simulink model "s_b16a4x32kf"  (R2018a)
settings: Solver=VariableStepDiscrete  StartTime=0.0  StopTime=1000  RelTol=1e-3
undefined symbols (not defined in the file): fft_stages, n_bits_ants, n_bits_xengs
libraries: xbsIndex_r4 x23740, casper_library_misc x48, casper_library_delays x8, xps_library x4, casper_library_scopes x1
(part 93 of 219)

== system s_b16a4x32kf/sys2/pkt_reord/munge/split ==
  bus_in : Inport
  reinterpret{1..9} (9 alike) : xbsIndex_r4/Reinterpret  force_arith_type=on  arith_type=Unsigned  force_bin_pt=on  bin_pt=0  block_type=reinterpret
  slice1 : xbsIndex_r4/Slice  nbits=32  boolean_output=off  mode=Upper Bit Location + Width  bit1=-225  base1=MSB of Input  bit0=0  base0=LSB of Input  dbl_ovrd=off  block_type=slice
  slice2 : xbsIndex_r4/Slice  nbits=32  boolean_output=off  mode=Upper Bit Location + Width  bit1=-193  base1=MSB of Input  bit0=0  base0=LSB of Input  dbl_ovrd=off  block_type=slice
  slice3 : xbsIndex_r4/Slice  nbits=32  boolean_output=off  mode=Upper Bit Location + Width  bit1=-161  base1=MSB of Input  bit0=0  base0=LSB of Input  dbl_ovrd=off  block_type=slice
  slice4 : xbsIndex_r4/Slice  nbits=32  boolean_output=off  mode=Upper Bit Location + Width  bit1=-129  base1=MSB of Input  bit0=0  base0=LSB of Input  dbl_ovrd=off  block_type=slice
  slice5 : xbsIndex_r4/Slice  nbits=32  boolean_output=off  mode=Upper Bit Location + Width  bit1=-97  base1=MSB of Input  bit0=0  base0=LSB of Input  dbl_ovrd=off  block_type=slice
  slice6 : xbsIndex_r4/Slice  nbits=32  boolean_output=off  mode=Upper Bit Location + Width  bit1=-65  base1=MSB of Input  bit0=0  base0=LSB of Input  dbl_ovrd=off  block_type=slice
  slice7 : xbsIndex_r4/Slice  nbits=32  boolean_output=off  mode=Upper Bit Location + Width  bit1=-33  base1=MSB of Input  bit0=0  base0=LSB of Input  dbl_ovrd=off  block_type=slice
  slice8 : xbsIndex_r4/Slice  nbits=32  boolean_output=off  mode=Upper Bit Location + Width  bit1=-1  base1=MSB of Input  bit0=0  base0=LSB of Input  dbl_ovrd=off  block_type=slice
  slice9 : xbsIndex_r4/Slice  nbits=1  boolean_output=off  mode=Upper Bit Location + Width  bit1=0  base1=MSB of Input  bit0=0  base0=LSB of Input  dbl_ovrd=off  block_type=slice
  msb_out9 : Outport
  out8 : Outport  Port=2
  out7 : Outport  Port=3
  out6 : Outport  Port=4
  out5 : Outport  Port=5
  out4 : Outport  Port=6
  out3 : Outport  Port=7
  out2 : Outport  Port=8
  lsb_out1 : Outport  Port=9
  wires:
  bus_in/1 -> slice9/1, slice8/1, slice7/1, slice6/1, slice5/1, slice4/1, slice3/1, slice2/1, slice1/1
  slice9/1 -> reinterpret9/1
  reinterpret9/1 -> msb_out9/1
  slice8/1 -> reinterpret8/1
  reinterpret8/1 -> out8/1
  slice7/1 -> reinterpret7/1
  reinterpret7/1 -> out7/1
  slice6/1 -> reinterpret6/1
  reinterpret6/1 -> out6/1
  slice5/1 -> reinterpret5/1
  reinterpret5/1 -> out5/1
  slice4/1 -> reinterpret4/1
  reinterpret4/1 -> out4/1
  slice3/1 -> reinterpret3/1
  reinterpret3/1 -> out3/1
  slice2/1 -> reinterpret2/1
  reinterpret2/1 -> out2/1
  slice1/1 -> reinterpret1/1
  reinterpret1/1 -> lsb_out1/1

== system s_b16a4x32kf/sys2/pkt_reord/munge1/join ==
  in1 : Inport
  in2 : Inport  Port=2
  concatenate : xbsIndex_r4/Concat  num_inputs=2  dbl_ovrd=off  block_type=concat
  reinterpret1 : xbsIndex_r4/Reinterpret  force_arith_type=on  arith_type=Unsigned  force_bin_pt=on  bin_pt=0  block_type=reinterpret
      settings: infoedit="Changes signal type without altering the binary representation.   You can changed the signal between signed and unsigned, and relocate the binary point.<br><br>Hardware notes: In hardware this block costs nothing.<br><br>Example:  Suppose the input is 6 bits wide, signed, with 2 fractional bits, and the output is forced to unsigned with 0 fractional bits.  Then an input of -2.0 (1110.00 in binary 2's complement) becomes an output of 56 (111000 in binary)."
  reinterpret2 : xbsIndex_r4/Reinterpret  force_arith_type=on  arith_type=Unsigned  force_bin_pt=on  bin_pt=0  block_type=reinterpret
      settings: infoedit="Changes signal type without altering the binary representation.   You can changed the signal between signed and unsigned, and relocate the binary point.<br><br>Hardware notes: In hardware this block costs nothing.<br><br>Example:  Suppose the input is 6 bits wide, signed, with 2 fractional bits, and the output is forced to unsigned with 0 fractional bits.  Then an input of -2.0 (1110.00 in binary 2's complement) becomes an output of 56 (111000 in binary)."
  bus_out : Outport
  wires:
  concatenate/1 -> bus_out/1
  in1/1 -> reinterpret1/1
  reinterpret1/1 -> concatenate/1
  in2/1 -> reinterpret2/1
  reinterpret2/1 -> concatenate/2

== system s_b16a4x32kf/sys2/pkt_reord/munge1/split ==
  bus_in : Inport
  reinterpret1 : xbsIndex_r4/Reinterpret  force_arith_type=on  arith_type=Unsigned  force_bin_pt=on  bin_pt=0  block_type=reinterpret
  reinterpret2 : xbsIndex_r4/Reinterpret  force_arith_type=on  arith_type=Unsigned  force_bin_pt=on  bin_pt=0  block_type=reinterpret
  slice1 : xbsIndex_r4/Slice  nbits=32  boolean_output=off  mode=Upper Bit Location + Width  bit1=-1  base1=MSB of Input  bit0=0  base0=LSB of Input  dbl_ovrd=off  block_type=slice
  slice2 : xbsIndex_r4/Slice  nbits=1  boolean_output=off  mode=Upper Bit Location + Width  bit1=0  base1=MSB of Input  bit0=0  base0=LSB of Input  dbl_ovrd=off  block_type=slice
  msb_out2 : Outport
  lsb_out1 : Outport  Port=2
  wires:
  bus_in/1 -> slice2/1, slice1/1
  slice2/1 -> reinterpret2/1
  reinterpret2/1 -> msb_out2/1
  slice1/1 -> reinterpret1/1
  reinterpret1/1 -> lsb_out1/1

== system s_b16a4x32kf/sys2/pkt_reord/output_control/edge_detect ==
  in : Inport
  Delay : xbsIndex_r4/Delay  rst=off  infoeditControl=Selection of Reset will increase slice count due to use of real FFs and instead of SRLs  en=off  latency=1  reg_retiming=on  dbl_ovrd=off  block_type=delay
      settings: xl_area=[0, 0, 0, 0, 0, 0, 0]
  Inverter : xbsIndex_r4/Inverter  en=off  latency=0  dbl_ovrd=off  block_type=inv
      settings: xl_area=[0, 0, 0, 0, 0, 0, 0]
  edge_op : xbsIndex_r4/Logical  logical_function=XNOR  inputs=2  en=off  latency=0  precision=Full  arith_type=Unsigned  n_bits=8  bin_pt=2  align_bp=on  dbl_ovrd=off  block_type=logical
      settings: xl_area=[0, 0, 0, 0, 0, 0, 0]
  out : Outport
  wires:
  Inverter/1 -> edge_op/1
  edge_op/1 -> out/1
  in/1 -> Inverter/1, Delay/1
  Delay/1 -> edge_op/2

== system s_b16a4x32kf/sys2/pkt_reord/output_control/edge_detect1 ==
  in : Inport
  Delay : xbsIndex_r4/Delay  rst=off  infoeditControl=Selection of Reset will increase slice count due to use of real FFs and instead of SRLs  en=off  latency=1  reg_retiming=on  dbl_ovrd=off  block_type=delay
      settings: xl_area=[0, 0, 0, 0, 0, 0, 0]
  Inverter : xbsIndex_r4/Inverter  en=off  latency=0  dbl_ovrd=off  block_type=inv
      settings: xl_area=[0, 0, 0, 0, 0, 0, 0]
  edge_op : xbsIndex_r4/Logical  logical_function=XNOR  inputs=2  en=off  latency=0  precision=Full  arith_type=Unsigned  n_bits=8  bin_pt=2  align_bp=on  dbl_ovrd=off  block_type=logical
      settings: xl_area=[0, 0, 0, 0, 0, 0, 0]
  out : Outport
  wires:
  Delay/1 -> edge_op/2
  in/1 -> Delay/1, Inverter/1
  edge_op/1 -> out/1
  Inverter/1 -> edge_op/1

== system s_b16a4x32kf/sys2/pkt_reord/output_control/pulse_ext ==
  in : Inport
  Constant5 : xbsIndex_r4/Constant  const=pulse_len-1  gui_display_data_type=Fixed-point  arith_type=Unsigned  n_bits=bits  bin_pt=0  preci_type=Single  exp_width=8  frac_width=24  explicit_period=off  period=1  equ=P=C  opselect=C  inp2=PCIN>>17  opr=+  inp1=P  carry=CIN  dbl_ovrd=off  block_type=constant
      settings: block_version=9.1.01
  Counter3 : xbsIndex_r4/Counter  cnt_type=Free Running  cnt_to=1023  operation=Up  start_count=0  cnt_by_val=1  arith_type=Unsigned  n_bits=bits  bin_pt=0  load_pin=off  rst=on  en=on  explicit_period=on  period=1  use_behavioral_HDL=off  implementation=Fabric  use_rpm=on  dbl_ovrd=off  block_type=counter
      settings: xl_area=[0, 0, 0, 0, 0, 0, 0]  block_version=9.1.01
  Relational5 : xbsIndex_r4/Relational  mode=a<=b  op_type=Bool  en=off  latency=0  dbl_ovrd=off  block_type=relational
      settings: xl_area=[0, 0, 0, 0, 0, 0, 0]  block_version=9.1.01
  posedge : Subsystem  Tag=Rising Edge Detector
  out : Outport
  wires:
  Counter3/1 -> Relational5/1
  Constant5/1 -> Relational5/2
  Relational5/1 -> Counter3/2, out/1
  in/1 -> posedge/1(In)
  posedge/1(Out) -> Counter3/1

== system s_b16a4x32kf/sys2/vacc/Subsystem/edge_detect2 ==
  in : Inport
  Delay : xbsIndex_r4/Delay  rst=off  infoeditControl=Selection of Reset will increase slice count due to use of real FFs and instead of SRLs  en=off  latency=1  reg_retiming=on  dbl_ovrd=off  block_type=delay
      settings: xl_area=[0, 0, 0, 0, 0, 0, 0]
  Inverter : xbsIndex_r4/Inverter  en=off  latency=0  dbl_ovrd=off  block_type=inv
      settings: xl_area=[0, 0, 0, 0, 0, 0, 0]
  edge_op : xbsIndex_r4/Logical  logical_function=NOR  inputs=2  en=off  latency=0  precision=Full  arith_type=Unsigned  n_bits=8  bin_pt=2  align_bp=on  dbl_ovrd=off  block_type=logical
      settings: xl_area=[0, 0, 0, 0, 0, 0, 0]
  out : Outport
  wires:
  Inverter/1 -> edge_op/1
  edge_op/1 -> out/1
  in/1 -> Inverter/1, Delay/1
  Delay/1 -> edge_op/2

== system s_b16a4x32kf/sys2/vacc/Subsystem/edge_detect6 ==
  in : Inport
  Delay : xbsIndex_r4/Delay  rst=off  infoeditControl=Selection of Reset will increase slice count due to use of real FFs and instead of SRLs  en=off  latency=1  reg_retiming=on  dbl_ovrd=off  block_type=delay
      settings: xl_area=[0, 0, 0, 0, 0, 0, 0]
  Inverter : xbsIndex_r4/Inverter  en=off  latency=0  dbl_ovrd=off  block_type=inv
      settings: xl_area=[0, 0, 0, 0, 0, 0, 0]
  edge_op : xbsIndex_r4/Logical  logical_function=AND  inputs=2  en=off  latency=0  precision=Full  arith_type=Unsigned  n_bits=8  bin_pt=2  align_bp=on  dbl_ovrd=off  block_type=logical
      settings: xl_area=[0, 0, 0, 0, 0, 0, 0]
  out : Outport
  wires:
  Delay/1 -> edge_op/2
  in/1 -> Delay/1, Inverter/1
  edge_op/1 -> out/1
  Inverter/1 -> edge_op/1

== system s_b16a4x32kf/sys2/vacc/hmc_vacc/acc ==
  a : Inport
  b : Inport  Port=2
  Slice2 : xbsIndex_r4/Slice  nbits=n_bits*n_inputs  boolean_output=off  mode=Lower Bit Location + Width  bit1=-32  base1=MSB of Input  bit0=0  base0=LSB of Input  dbl_ovrd=off  block_type=slice
      settings: block_version=9.2.01
  Slice3 : xbsIndex_r4/Slice  nbits=n_bits*n_inputs  boolean_output=off  mode=Lower Bit Location + Width  bit1=-32  base1=MSB of Input  bit0=0  base0=LSB of Input  dbl_ovrd=off  block_type=slice
      settings: block_version=9.2.01
  bus_addsub : Subsystem  Tag=cmac_delinked  mask(bus_addsub){opmode=0, n_bits_a=repmat(n_bits, 1, n_inputs), bin_pt_a=0, type_a=1, n_bits_b=repmat(n_bits, 1, n_inputs), bin_pt_b=0, type_b=1, cmplx=off, misc=off, async=off, floating_point=off, float_type=single, exp_width=6, frac_width=19, n_bits_out=n_bits, bin_pt_out=0, type_out=1, quantization=0, overflow=1, add_implementation=fabric core, csp_latency=2, pipeline_en=off, pipeline_latency=0}
      mask prompts: opmode "mode (Addition=0, Subtraction=1)"; n_bits_a "a input bit widths"; bin_pt_a "a input binary points"; type_a "a input type (Unsigned=0, Signed=1)"; n_bits_b "b input bit widths"; bin_pt_b "b input binary points"; type_b "b input type (Unsigned=0, Signed=1)"; cmplx "complex"; misc "misc support"; async "asynchronous operation"; floating_point "floating point"; exp_width "exponent width"; frac_width "fraction width"; n_bits_out "output bit widths"; bin_pt_out "output binary points"; type_out "output type (Unsigned=0, Signed=1)"; quantization "quantization strategy (Truncate=0, Round  (unbiased: +/- Inf)=1)"; overflow "overflow strategy (Wrap=0, Saturate=1, Flag as error=2)"; add_implementation "adder implementation"; csp_latency "latency"; pipeline_en "pipeline enable"; pipeline_latency "pipeline latency"
      mask help: Add/subtract components of two busses
      mask init: same as s_b16a4x32kf/bus_addsub
      mask Callback floating_point:
      | onoff = get_param(gcb, 'floating_point');
      | if strcmp(onoff,'on')
      |     enable_fixpt = 'off'
      |     set_param_state(gcb, 'float_type', 'on')
      | 
      |     f_type = get_param(gcb, 'float_type')
      |     if strcmp(f_type,'custom')
      |         set_param_state(gcb, 'exp_width', 'on')
      |         set_param_state(gcb, 'frac_width', 'on')
      |     else
      |         set_param_state(gcb, 'exp_width', 'off')
      |         set_param_state(gcb, 'frac_width', 'off')
      |     end
      | 
      | 
      | else
      |     enable_fixpt = 'on'
      |     set_param_state(gcb, 'float_type', 'off')
      |     set_param_state(gcb, 'exp_width', 'off')
      |     set_param_state(gcb, 'frac_width', 'off')
      | end
      | 
      | set_param_state(gcb, 'n_bits_a', enable_fixpt)
      | set_param_state(gcb, 'bin_pt_a', enable_fixpt)
      | set_param_state(gcb, 'type_a', enable_fixpt)
      | set_param_state(gcb, 'n_bits_b', enable_fixpt)
      | set_param_state(gcb, 'bin_pt_b', enable_fixpt)
      | set_param_state(gcb, 'type_b', enable_fixpt)
      | 
      | set_param_state(gcb, 'n_bits_out', enable_fixpt)
      | set_param_state(gcb, 'bin_pt_out', enable_fixpt)
      | set_param_state(gcb, 'type_out', enable_fixpt)
      | set_param_state(gcb, 'quantization', enable_fixpt)
      | set_param_state(gcb, 'overflow', enable_fixpt)
      mask TypeOptions float_type: single | custom
      mask Callback float_type:
      | f_type = get_param(gcb, 'float_type')
      | if strcmp(f_type,'custom')
      |     set_param_state(gcb, 'exp_width', 'on')
      |     set_param_state(gcb, 'frac_width', 'on')
      | else
      |     set_param_state(gcb, 'exp_width', 'off')
      |     set_param_state(gcb, 'frac_width', 'off')
      | end
      mask TypeOptions add_implementation: behavioral HDL | fabric core | DSP48 core
  Out : Outport
  wires:
  a/1 -> Slice3/1
  Slice3/1 -> bus_addsub/1(a)
  Slice2/1 -> bus_addsub/2(b)
  bus_addsub/1(dout) -> Out/1
  b/1 -> Slice2/1

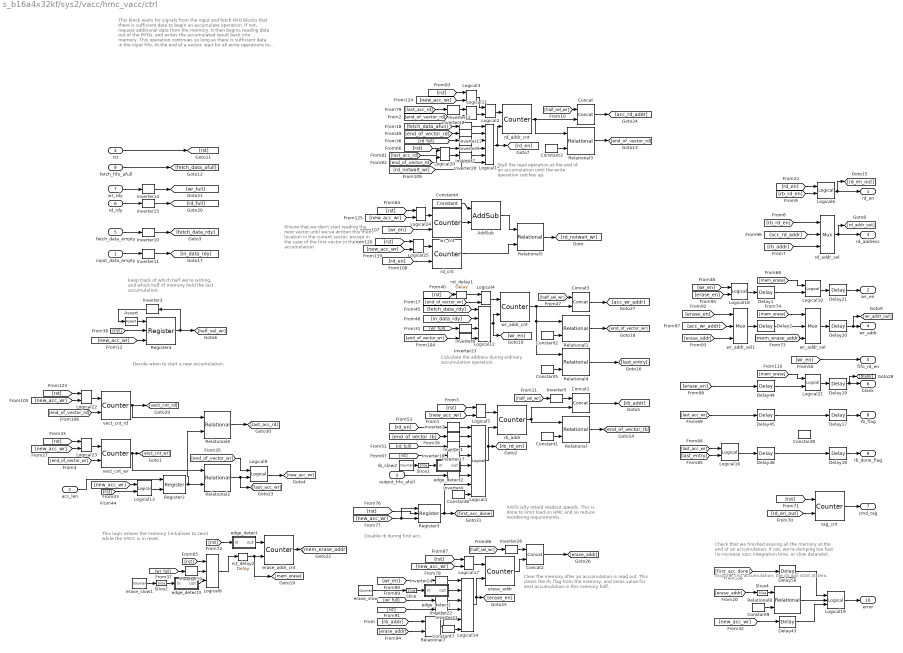
== system s_b16a4x32kf/sys2/vacc/hmc_vacc/ctrl ==
  note: Clear the memory after an accumulation is read out.
      | This clears the rb_flag from the memory, and
      | zeros value for next accumulation in this memory half.
  note: Stall the read operation
      | at the end of an accumulation
      | until the write operation catches up.
  note: Ensure that we don't start reading
      | the next vector until we've written
      | this mem location in the current vector,
      | except in the case of the first vector in
      | the accumulation.
  note: Disable rb during first acc.
  note: Artificially retard readout speeds.
      | This is done to limit load on HMC and
      | so reduce reordering requirements.
  note: This logic erases the memory (initialises to zero)
      | while the VACC is in reset.
  note: Decide when to start a new accumulation.
  note: Calculate the address during ordinary
      | accumulation operation.
  note: keep track of which half we're writing,
      | and which half of memory
      | held the last accumulation.
  note: This block waits for signals from the
      | input and fetch FIFO blocks that there is sufficient data
      | to begin an accumulate operation.
      |
      | If not, request additional data from the memory.
      |
      | It then begins reading data out of the FIFOs, and writes the
      | accumulated result back into memory.
      |
      | This operation continues so long as there is
      | sufficient data in the input fifo.
      |
      | At the end of a vector, wait for all write operations
      | to finish before starting the next vector.
      |
      | Simultaneously, read back the previous integration during
      | unused rd/write operations. After reading a previous accumulated
      | value, try to clear that memory location.
  note: Check that we finished erasing all the memory
      | at the end of an accumulation.
      | If not, we're dumping too fast
      | (ie increase vacc integration time, or slow datarate).
  note: skip the first accumulation; the ctr will start at zero.
  input_data_empty : Inport
  acc_len : Inport  Port=2
  output_fifo_afull : Inport  Port=3
  rst : Inport  Port=4
  fetch_data_empty : Inport  Port=5
  rd_rdy : Inport  Port=6
  wr_rdy : Inport  Port=7
  fetch_fifo_afull : Inport  Port=8
  AddSub : xbsIndex_r4/AddSub  mode=Addition  use_carryin=off  use_carryout=off  en=off  latency=1  precision=Full  arith_type=Unsigned  n_bits=16  bin_pt=14  quantization=Truncate  overflow=Wrap  use_behavioral_HDL=off  hw_selection=Fabric  pipelined=off  dbl_ovrd=off  block_type=addsub
  Assert : xbsIndex_r4/Assert  assert_type=on  type_source=Explicitly  gui_display_data_type=Fixed-point  arith_type=Unsigned  n_bits=1  bin_pt=0  preci_type=Single  exp_width=8  frac_width=24  assert_rate=on  rate_source=Explicitly  period=1  output_port=on  block_type=assert
      settings: infoedit=Asserts a user-defined sample rate and/or type on a signal.<P><P>Hardware notes: In hardware this block costs nothing.  block_version=10.1.3
  Concat{,1..3} (4 alike) : xbsIndex_r4/Concat  num_inputs=2  dbl_ovrd=off  block_type=concat
      settings: block_version=10.1.3
  Constant{1..3,9} (4 alike) : xbsIndex_r4/Constant  const=vector_len  gui_display_data_type=Fixed-point  arith_type=Unsigned  n_bits=vector_bits  bin_pt=0  preci_type=Single  exp_width=8  frac_width=24  explicit_period=on  period=1  equ=P=C  opselect=C  inp2=PCIN>>17  opr=+  inp1=P  carry=CIN  dbl_ovrd=off  block_type=constant
  Constant4 : xbsIndex_r4/Constant  const=vector_len-4  gui_display_data_type=Fixed-point  arith_type=Unsigned  n_bits=vector_bits  bin_pt=0  preci_type=Single  exp_width=8  frac_width=24  explicit_period=on  period=1  equ=P=C  opselect=C  inp2=PCIN>>17  opr=+  inp1=P  carry=CIN  dbl_ovrd=off  block_type=constant
  Constant5 : xbsIndex_r4/Constant  const=vector_len-1  gui_display_data_type=Fixed-point  arith_type=Unsigned  n_bits=vector_bits  bin_pt=0  preci_type=Single  exp_width=8  frac_width=24  explicit_period=on  period=1  equ=P=C  opselect=C  inp2=PCIN>>17  opr=+  inp1=P  carry=CIN  dbl_ovrd=off  block_type=constant
  Constant6 : xbsIndex_r4/Constant  const=1  gui_display_data_type=Boolean  arith_type=Boolean  n_bits=1  bin_pt=0  preci_type=Single  exp_width=8  frac_width=24  explicit_period=on  period=1  equ=P=C  opselect=C  inp2=PCIN>>17  opr=+  inp1=P  carry=CIN  dbl_ovrd=off  block_type=constant
  Constant7 : xbsIndex_r4/Constant  const=1  gui_display_data_type=Boolean  arith_type=Boolean  n_bits=1  bin_pt=0  preci_type=Single  exp_width=8  frac_width=24  explicit_period=on  period=1  equ=P=C  opselect=C  inp2=PCIN>>17  opr=+  inp1=P  carry=CIN  dbl_ovrd=off  block_type=constant
  Constant8 : xbsIndex_r4/Constant  const=0  gui_display_data_type=Boolean  arith_type=Boolean  n_bits=1  bin_pt=0  preci_type=Single  exp_width=8  frac_width=24  explicit_period=on  period=1  equ=P=C  opselect=C  inp2=PCIN>>17  opr=+  inp1=P  carry=CIN  dbl_ovrd=off  block_type=constant
  Delay{1..2,44..46} (5 alike) : xbsIndex_r4/Delay  rst=off  infoeditControl=Selection of Reset will increase slice count due to use of real FFs and instead of SRLs  en=off  latency=delay_fifo  reg_retiming=on  dbl_ovrd=off  block_type=delay
      settings: infoedit=Hardware notes: A delay line is a chain, each link of which is an SRL16 or SRL32 followed by a flip-flop.
  Delay{17..21} (5 alike) : xbsIndex_r4/Delay  rst=off  infoeditControl=Selection of Reset will increase slice count due to use of real FFs and instead of SRLs  en=off  latency=delay_adder  reg_retiming=on  dbl_ovrd=off  block_type=delay
      settings: infoedit=Hardware notes: A delay line is a chain, each link of which is an SRL16 or SRL32 followed by a flip-flop.
  Delay43 : xbsIndex_r4/Delay  rst=off  infoeditControl=Selection of Reset will increase slice count due to use of real FFs and instead of SRLs  en=off  latency=1  reg_retiming=on  dbl_ovrd=off  block_type=delay
      settings: infoedit=Hardware notes: A delay line is a chain, each link of which is an SRL16 or SRL32 followed by a flip-flop.
  Delay56 : xbsIndex_r4/Delay  rst=off  infoeditControl=Selection of Reset will increase slice count due to use of real FFs and instead of SRLs  en=off  latency=1  reg_retiming=on  dbl_ovrd=off  block_type=delay
      settings: infoedit=Hardware notes: A delay line is a chain, each link of which is an SRL16 or SRL32 followed by a flip-flop.
  Inverter{1..5,7..24,26} (24 alike) : xbsIndex_r4/Inverter  en=off  latency=0  dbl_ovrd=off  block_type=inv
  Logical1 : xbsIndex_r4/Logical  logical_function=AND  inputs=8  en=off  latency=0  precision=Full  arith_type=Unsigned  n_bits=16  bin_pt=0  align_bp=on  dbl_ovrd=off  block_type=logical
  Logical{2..6,10,13,17..18,21..25} (14 alike) : xbsIndex_r4/Logical  logical_function=OR  inputs=2  en=off  latency=0  precision=Full  arith_type=Unsigned  n_bits=16  bin_pt=0  align_bp=on  dbl_ovrd=off  block_type=logical
  Logical{9,11,16,20} (4 alike) : xbsIndex_r4/Logical  logical_function=AND  inputs=2  en=off  latency=0  precision=Full  arith_type=Unsigned  n_bits=16  bin_pt=0  align_bp=on  dbl_ovrd=off  block_type=logical
  Logical12 : xbsIndex_r4/Logical  logical_function=AND  inputs=4  en=off  latency=0  precision=Full  arith_type=Unsigned  n_bits=16  bin_pt=0  align_bp=on  dbl_ovrd=off  block_type=logical
  Logical14 : xbsIndex_r4/Logical  logical_function=AND  inputs=6  en=off  latency=0  precision=Full  arith_type=Unsigned  n_bits=16  bin_pt=0  align_bp=on  dbl_ovrd=off  block_type=logical
  Logical15 : xbsIndex_r4/Logical  logical_function=AND  inputs=6  en=off  latency=0  precision=Full  arith_type=Unsigned  n_bits=16  bin_pt=0  align_bp=on  dbl_ovrd=off  block_type=logical
  Logical19 : xbsIndex_r4/Logical  logical_function=AND  inputs=3  en=off  latency=0  precision=Full  arith_type=Unsigned  n_bits=16  bin_pt=0  align_bp=on  dbl_ovrd=off  block_type=logical
  Logical8 : xbsIndex_r4/Logical  logical_function=AND  inputs=3  en=off  latency=0  precision=Full  arith_type=Unsigned  n_bits=16  bin_pt=0  align_bp=on  dbl_ovrd=off  block_type=logical
  Register2 : xbsIndex_r4/Register  init=0  rst=off  en=on  dbl_ovrd=off  block_type=register
  Register3 : xbsIndex_r4/Register  init=0  rst=on  en=on  dbl_ovrd=off  block_type=register
  Register4 : xbsIndex_r4/Register  init=0  rst=on  en=on  dbl_ovrd=off  block_type=register
  Relational{,1..4,6} (6 alike) : xbsIndex_r4/Relational  mode=a>=b  op_type=Bool  en=off  latency=0  dbl_ovrd=off  block_type=relational
      settings: block_version=10.1.3
  Relational5 : xbsIndex_r4/Relational  mode=a>b  op_type=Bool  en=off  latency=1  dbl_ovrd=off  block_type=relational
      settings: block_version=10.1.3
  Relational7 : xbsIndex_r4/Relational  mode=a>b  op_type=Bool  en=off  latency=0  dbl_ovrd=off  block_type=relational
      settings: block_version=10.1.3
  Relational8 : xbsIndex_r4/Relational  mode=a!=b  op_type=Bool  en=off  latency=1  dbl_ovrd=off  block_type=relational
      settings: block_version=10.1.3
  Slice : xbsIndex_r4/Slice  nbits=1  boolean_output=on  mode=Upper Bit Location + Width  bit1=0  base1=MSB of Input  bit0=0  base0=LSB of Input  dbl_ovrd=off  block_type=slice
  Slice1 : xbsIndex_r4/Slice  nbits=1  boolean_output=on  mode=Upper Bit Location + Width  bit1=0  base1=MSB of Input  bit0=0  base0=LSB of Input  dbl_ovrd=off  block_type=slice
  Slice2 : xbsIndex_r4/Slice  nbits=1  boolean_output=on  mode=Upper Bit Location + Width  bit1=0  base1=MSB of Input  bit0=0  base0=LSB of Input  dbl_ovrd=off  block_type=slice
  Slice4 : xbsIndex_r4/Slice  nbits=1  boolean_output=off  mode=Two Bit Locations  bit1=-1  base1=MSB of Input  bit0=0  base0=LSB of Input  dbl_ovrd=off  block_type=slice
  edge_detect : Subsystem  mask(edge_detect){edge=Rising, polarity=Active High, x_in=[0 0.08 0.08 0.16 0.16 0.24 0.24 0.32 0.32 0.4], y_in=[-1 -1  1  1  1  1  1  1  1  1], x_out=[0.6 0.68 0.68 0.76 0.76 0.84 0.84 0.92 0.92 1], y_out=[-1 -1  1  1 -1 -1 -1 -1 -1 -1]}
      mask prompts: edge "Edge Type"; polarity "Output Polarity"; x_in "Input X Positions"; y_in "Input Y Positions"; x_out "Output X Positions"; y_out "Output Y Positions"
      mask help: Output is active for one-cycle after each edge of the specified type (i.e. rising, falling or both).
      mask init: same as s_b16a4x32kf/edge_detect
      settings: AttributesFormatString=|
      | rising edges
      | active high
      mask Help: Output is active for one-cycle after each edge of the specified type (i.e. rising, falling, or both).  Latency is zero.
      mask TypeOptions edge: Rising | Falling | Both
      mask TypeOptions polarity: Active High | Active Low
      mask Display:
      | plot(x_in_num,0.5+y_in_num*0.2);
      | plot(x_out_num,0.5+y_out_num*0.2);
  edge_detect1 : Subsystem  mask(edge_detect){edge=Rising, polarity=Active High, x_in=[0 0.08 0.08 0.16 0.16 0.24 0.24 0.32 0.32 0.4], y_in=[-1 -1  1  1  1  1  1  1  1  1], x_out=[0.6 0.68 0.68 0.76 0.76 0.84 0.84 0.92 0.92 1], y_out=[-1 -1  1  1 -1 -1 -1 -1 -1 -1]}
      mask prompts: edge "Edge Type"; polarity "Output Polarity"; x_in "Input X Positions"; y_in "Input Y Positions"; x_out "Output X Positions"; y_out "Output Y Positions"
      mask help: Output is active for one-cycle after each edge of the specified type (i.e. rising, falling or both).
      mask init: same as s_b16a4x32kf/edge_detect
      settings: AttributesFormatString=|
      | rising edges
      | active high
      mask Help: Output is active for one-cycle after each edge of the specified type (i.e. rising, falling, or both).  Latency is zero.
      mask TypeOptions edge: Rising | Falling | Both
      mask TypeOptions polarity: Active High | Active Low
      mask Display:
      | plot(x_in_num,0.5+y_in_num*0.2);
      | plot(x_out_num,0.5+y_out_num*0.2);
  edge_detect2 : Subsystem  mask(edge_detect){edge=Rising, polarity=Active High, x_in=[0 0.08 0.08 0.16 0.16 0.24 0.24 0.32 0.32 0.4], y_in=[-1 -1  1  1  1  1  1  1  1  1], x_out=[0.6 0.68 0.68 0.76 0.76 0.84 0.84 0.92 0.92 1], y_out=[-1 -1  1  1 -1 -1 -1 -1 -1 -1]}
      mask prompts: edge "Edge Type"; polarity "Output Polarity"; x_in "Input X Positions"; y_in "Input Y Positions"; x_out "Output X Positions"; y_out "Output Y Positions"
      mask help: Output is active for one-cycle after each edge of the specified type (i.e. rising, falling or both).
      mask init: same as s_b16a4x32kf/edge_detect
      settings: AttributesFormatString=|
      | rising edges
      | active high
      mask Help: Output is active for one-cycle after each edge of the specified type (i.e. rising, falling, or both).  Latency is zero.
      mask TypeOptions edge: Rising | Falling | Both
      mask TypeOptions polarity: Active High | Active Low
      mask Display:
      | plot(x_in_num,0.5+y_in_num*0.2);
      | plot(x_out_num,0.5+y_out_num*0.2);
  edge_detect3 : Subsystem  mask(edge_detect){edge=Rising, polarity=Active High, x_in=[0 0.08 0.08 0.16 0.16 0.24 0.24 0.32 0.32 0.4], y_in=[-1 -1  1  1  1  1  1  1  1  1], x_out=[0.6 0.68 0.68 0.76 0.76 0.84 0.84 0.92 0.92 1], y_out=[-1 -1  1  1 -1 -1 -1 -1 -1 -1]}
      mask prompts: edge "Edge Type"; polarity "Output Polarity"; x_in "Input X Positions"; y_in "Input Y Positions"; x_out "Output X Positions"; y_out "Output Y Positions"
      mask help: Output is active for one-cycle after each edge of the specified type (i.e. rising, falling or both).
      mask init: same as s_b16a4x32kf/edge_detect
      settings: AttributesFormatString=|
      | rising edges
      | active high
      mask Help: Output is active for one-cycle after each edge of the specified type (i.e. rising, falling, or both).  Latency is zero.
      mask TypeOptions edge: Rising | Falling | Both
      mask TypeOptions polarity: Active High | Active Low
      mask Display:
      | plot(x_in_num,0.5+y_in_num*0.2);
      | plot(x_out_num,0.5+y_out_num*0.2);
  erase_addr : xbsIndex_r4/Counter  cnt_type=Free Running  cnt_to=Inf  operation=Up  start_count=0  cnt_by_val=1  arith_type=Unsigned  n_bits=vector_bits  bin_pt=0  load_pin=off  rst=on  en=on  explicit_period=on  period=1  use_behavioral_HDL=off  implementation=Fabric  use_rpm=off  dbl_ovrd=off  block_type=counter
  erase_addr_cnt : xbsIndex_r4/Counter  cnt_type=Free Running  cnt_to=vector_len-1  operation=Up  start_count=0  cnt_by_val=1  arith_type=Unsigned  n_bits=vector_bits+1  bin_pt=0  load_pin=off  rst=on  en=on  explicit_period=on  period=1  use_behavioral_HDL=off  implementation=Fabric  use_rpm=off  dbl_ovrd=off  block_type=counter
  erase_slow : xbsIndex_r4/Counter  cnt_type=Free Running  cnt_to=Inf  operation=Up  start_count=0  cnt_by_val=1  arith_type=Unsigned  n_bits=4  bin_pt=0  load_pin=off  rst=off  en=off  explicit_period=on  period=1  use_behavioral_HDL=on  implementation=Fabric  use_rpm=off  dbl_ovrd=off  block_type=counter
  erase_slow1 : xbsIndex_r4/Counter  cnt_type=Free Running  cnt_to=Inf  operation=Up  start_count=0  cnt_by_val=1  arith_type=Unsigned  n_bits=2  bin_pt=0  load_pin=off  rst=off  en=off  explicit_period=on  period=1  use_behavioral_HDL=on  implementation=Fabric  use_rpm=off  dbl_ovrd=off  block_type=counter
  rb_addr : xbsIndex_r4/Counter  cnt_type=Free Running  cnt_to=Inf  operation=Up  start_count=0  cnt_by_val=1  arith_type=Unsigned  n_bits=vector_bits  bin_pt=0  load_pin=off  rst=on  en=on  explicit_period=on  period=1  use_behavioral_HDL=off  implementation=Fabric  use_rpm=off  dbl_ovrd=off  block_type=counter
  rb_slow2 : xbsIndex_r4/Counter  cnt_type=Free Running  cnt_to=Inf  operation=Up  start_count=0  cnt_by_val=1  arith_type=Unsigned  n_bits=4  bin_pt=0  load_pin=off  rst=off  en=off  explicit_period=on  period=1  use_behavioral_HDL=on  implementation=Fabric  use_rpm=off  dbl_ovrd=off  block_type=counter
  rd_addr_cnt : xbsIndex_r4/Counter  cnt_type=Free Running  cnt_to=vector_len-1  operation=Up  start_count=0  cnt_by_val=1  arith_type=Unsigned  n_bits=vector_bits  bin_pt=0  load_pin=off  rst=on  en=on  explicit_period=on  period=1  use_behavioral_HDL=off  implementation=Fabric  use_rpm=off  dbl_ovrd=off  block_type=counter
  rd_addr_sel : xbsIndex_r4/Mux  inputs=2  en=off  latency=0  precision=Full  arith_type=Unsigned  n_bits=16  bin_pt=14  quantization=Truncate  overflow=Wrap  dbl_ovrd=off  block_type=mux
  rd_cnt : xbsIndex_r4/Counter  cnt_type=Free Running  cnt_to=vector_len-1  operation=Up  start_count=0  cnt_by_val=1  arith_type=Unsigned  n_bits=vector_bits+22  bin_pt=0  load_pin=off  rst=on  en=on  explicit_period=on  period=1  use_behavioral_HDL=off  implementation=Fabric  use_rpm=off  dbl_ovrd=off  block_type=counter
  rst_delay1 : xbsIndex_r4/Delay  rst=off  infoeditControl=Selection of Reset will increase slice count due to use of real FFs and instead of SRLs  en=off  latency=2  reg_retiming=on  dbl_ovrd=off  block_type=delay
  rst_delay2 : xbsIndex_r4/Delay  rst=off  infoeditControl=Selection of Reset will increase slice count due to use of real FFs and instead of SRLs  en=off  latency=1  reg_retiming=on  dbl_ovrd=off  block_type=delay
      settings: infoedit=Hardware notes: A delay line is a chain, each link of which is an SRL16 or SRL32 followed by a flip-flop.
  tag_cnt : xbsIndex_r4/Counter  cnt_type=Free Running  cnt_to=Inf  operation=Up  start_count=0  cnt_by_val=1  arith_type=Unsigned  n_bits=9  bin_pt=0  load_pin=off  rst=on  en=on  explicit_period=on  period=1  use_behavioral_HDL=off  implementation=Fabric  use_rpm=off  dbl_ovrd=off  block_type=counter
  vect_cnt_rd : xbsIndex_r4/Counter  cnt_type=Free Running  cnt_to=Inf  operation=Up  start_count=1  cnt_by_val=1  arith_type=Unsigned  n_bits=32  bin_pt=0  load_pin=off  rst=on  en=on  explicit_period=on  period=1  use_behavioral_HDL=off  implementation=Fabric  use_rpm=off  dbl_ovrd=off  block_type=counter
  vect_cnt_wr : xbsIndex_r4/Counter  cnt_type=Free Running  cnt_to=Inf  operation=Up  start_count=1  cnt_by_val=1  arith_type=Unsigned  n_bits=32  bin_pt=0  load_pin=off  rst=on  en=on  explicit_period=on  period=1  use_behavioral_HDL=off  implementation=Fabric  use_rpm=off  dbl_ovrd=off  block_type=counter
  wr_addr_cnt : xbsIndex_r4/Counter  cnt_type=Free Running  cnt_to=vector_len-1  operation=Up  start_count=0  cnt_by_val=1  arith_type=Unsigned  n_bits=vector_bits  bin_pt=0  load_pin=off  rst=on  en=on  explicit_period=on  period=1  use_behavioral_HDL=off  implementation=Fabric  use_rpm=off  dbl_ovrd=off  block_type=counter
  wr_addr_sel : xbsIndex_r4/Mux  inputs=2  en=off  latency=0  precision=Full  arith_type=Unsigned  n_bits=16  bin_pt=14  quantization=Truncate  overflow=Wrap  dbl_ovrd=off  block_type=mux
  wr_addr_sel1 : xbsIndex_r4/Mux  inputs=2  en=off  latency=0  precision=Full  arith_type=Unsigned  n_bits=16  bin_pt=14  quantization=Truncate  overflow=Wrap  dbl_ovrd=off  block_type=mux
  wr_cnt : xbsIndex_r4/Counter  cnt_type=Free Running  cnt_to=vector_len-1  operation=Up  start_count=0  cnt_by_val=1  arith_type=Unsigned  n_bits=vector_bits+22  bin_pt=0  load_pin=off  rst=on  en=on  explicit_period=on  period=1  use_behavioral_HDL=off  implementation=Fabric  use_rpm=off  dbl_ovrd=off  block_type=counter
  rd_en : Outport
  wr_en : Outport  Port=2
  rd_address : Outport  Port=3
  wr_addr : Outport  Port=4
  fifo_rd_en : Outport  Port=5
  blank : Outport  Port=6
  cmd_tag : Outport  Port=7
  rb_flag : Outport  Port=8
  rb_done_flag : Outport  Port=9
  error : Outport  Port=10
  wires:
  Concat1/1 -> [rb_addr]
  rb_addr/1 -> Concat1/2, Relational/1
  [rb_addr] -> rd_addr_sel/3
  Inverter5/1 -> Concat1/1
  [half_sel_wr] -> Inverter5/1
  [half_sel_wr] -> Concat/1
  Register2/1 -> Relational6/2, Relational2/2
  Logical9/1 -> [new_acc_wr]
  rst/1 -> [rst]
  Constant3/1 -> Relational3/2
  Assert/1 -> Register4/1
  Inverter3/1 -> Assert/1
  Register4/1 -> [half_sel_wr], Inverter3/1
  rd_addr_sel/1 -> rd_address/1, [rd_addr_out]
  [rb_rd_en] -> Logical6/2
  Concat/1 -> [acc_rd_addr]
  [rb_rd_en] -> rd_addr_sel/1
  Logical6/1 -> rd_en/1, [rd_en_out]
  Relational/1 -> [end_of_vector_rb]
  rd_addr_cnt/1 -> Relational3/1, Concat/2
  Logical15/1 -> rd_addr_cnt/2, [rd_en]
  [end_of_vector_wr] -> vect_cnt_wr/2
  Logical2/1 -> rd_addr_cnt/1
  Logical3/1 -> Logical2/1
  Relational2/1 -> [last_acc_wr], Logical9/2
  [end_of_vector_wr] -> Logical9/1
  Logical1/1 -> rb_addr/2, [rb_rd_en]
  [rst] -> Register4/2
  [rd_en] -> Inverter2/1
  [new_acc_wr] -> Logical13/1
  [rst] -> Logical13/2
  acc_len/1 -> Register2/1
  Logical13/1 -> Register2/2
  Logical4/1 -> wr_addr_cnt/1
  fetch_data_empty/1 -> Inverter10/1
  input_data_empty/1 -> Inverter11/1
  Inverter10/1 -> [fetch_data_rdy]
  Inverter11/1 -> [in_data_rdy]
  [fetch_data_afull] -> Inverter12/1
  [end_of_vector_rd] -> Inverter13/1
  Inverter12/1 -> Logical15/1
  Inverter13/1 -> Logical15/2
  Relational1/1 -> [end_of_vector_wr]
  Constant2/1 -> Relational1/2
  [end_of_vector_wr] -> Logical4/2
  [rst] -> rst_delay1/1
  [fetch_data_rdy] -> Logical12/1
  [in_data_rdy] -> Logical12/2
  Logical12/1 -> wr_addr_cnt/2, [wr_en]
  [half_sel_wr] -> Concat3/1
  wr_addr_cnt/1 -> Concat3/2, Relational1/1, Relational4/1
  [rd_en] -> Logical6/1
  [wr_en] -> fifo_rd_en/1
  Constant1/1 -> Relational/2
  [end_of_vector_rb] -> Inverter1/1
  rd_rdy/1 -> Inverter15/1
  wr_rdy/1 -> Inverter14/1
  [wr_full] -> Inverter8/1
  Inverter8/1 -> Logical12/3
  [rd_full] -> Inverter9/1
  Inverter14/1 -> [wr_full]
  Inverter15/1 -> [rd_full]
  Delay2/1 -> wr_addr_sel/2
  [rd_full] -> Inverter17/1
  output_fifo_afull/1 -> Inverter4/1
  fetch_fifo_afull/1 -> [fetch_data_afull]
  Inverter17/1 -> Logical1/3
  Inverter2/1 -> Logical1/1
  Inverter1/1 -> Logical1/2
  Inverter9/1 -> Logical15/3
  Constant5/1 -> Relational4/2
  Relational4/1 -> [last_entry]
  [new_acc_wr] -> Logical5/2
  [rst] -> Logical5/1
  Logical5/1 -> rb_addr/1
  [rst] -> Inverter7/1
  Inverter7/1 -> Logical15/4
  [rst] -> Inverter16/1
  edge_detect2/1(out) -> Logical1/5
  Inverter16/1 -> Logical1/4
  [rd_en_out] -> tag_cnt/2
  tag_cnt/1 -> cmd_tag/1
  rst_delay1/1 -> Logical4/1
  [rst] -> Logical8/1
  [wr_full] -> Inverter19/1
  Inverter19/1 -> Logical8/2
  Logical8/1 -> rst_delay2/1
  rst_delay2/1 -> erase_addr_cnt/2, [mem_erase]
  [rst] -> edge_detect/1(in)
  edge_detect/1(out) -> erase_addr_cnt/1
  wr_addr_sel/1 -> Delay20/1
  erase_addr_cnt/1 -> [mem_erase_addr]
  [mem_erase_addr] -> wr_addr_sel/3
  [mem_erase] -> wr_addr_sel/1
  Logical10/1 -> Delay21/1
  Delay1/1 -> Logical10/2
  [mem_erase] -> Logical10/1
  Inverter4/1 -> Logical1/6
  [rst] -> Register3/2
  [new_acc_wr] -> Register3/3, Register3/1
  vect_cnt_wr/1 -> Relational2/1, [vect_cnt_wr]
  [last_acc_wr] -> Logical16/1
  [last_entry] -> Logical16/2
  Delay17/1 -> rb_flag/1
  Delay18/1 -> rb_done_flag/1
  Concat2/1 -> [erase_addr]
  erase_addr/1 -> Concat2/2
  Inverter26/1 -> Concat2/1
  [half_sel_wr] -> Inverter26/1
  Logical14/1 -> [erase_en], erase_addr/2
  [wr_en] -> Inverter24/1
  [wr_full] -> Inverter22/1
  Inverter22/1 -> Logical14/3
  Inverter24/1 -> Logical14/1
  [new_acc_wr] -> Logical17/2
  [rst] -> Logical17/1
  Logical17/1 -> erase_addr/1
  [rst] -> Inverter21/1
  Relational7/1 -> Logical14/5
  Inverter21/1 -> Logical14/4
  Slice/1 -> edge_detect1/1(in)
  [rb_addr] -> Relational7/1
  [erase_addr] -> Relational7/2
  wr_addr_sel1/1 -> Delay2/1
  [erase_en] -> wr_addr_sel1/1
  [erase_addr] -> wr_addr_sel1/3
  edge_detect1/1(out) -> Logical14/2
  [wr_en] -> Logical18/1
  [erase_en] -> Logical18/2
  Logical18/1 -> Delay1/1
  [acc_rd_addr] -> rd_addr_sel/2
  Concat3/1 -> [acc_wr_addr]
  [acc_wr_addr] -> wr_addr_sel1/2
  [erase_en] -> Delay44/1
  Register3/1 -> [first_acc_done], Logical1/7
  Delay20/1 -> wr_addr/1, [wr_addr_out]
  Delay21/1 -> wr_en/1
  rb_slow2/1 -> Slice1/1
  Slice1/1 -> edge_detect2/1(in)
  [last_acc_rd] -> Inverter18/1
  Inverter18/1 -> Logical11/1
  [end_of_vector_rd] -> Logical11/2
  Logical11/1 -> Logical2/2
  [end_of_vector_rd] -> Logical20/2
  [last_acc_rd] -> Logical20/1
  Logical20/1 -> Inverter20/1
  Inverter20/1 -> Logical15/5
  [end_of_vector_wr] -> Inverter23/1
  Inverter23/1 -> Logical12/4
  erase_slow/1 -> Slice/1
  Slice2/1 -> edge_detect3/1(in)
  erase_slow1/1 -> Slice2/1
  edge_detect3/1(out) -> Logical8/3
  Relational3/1 -> [end_of_vector_rd]
  [rd_notwait_wr] -> Logical15/6
  rd_cnt/1 -> Relational5/2
  Relational5/1 -> [rd_notwait_wr]
  Logical25/1 -> rd_cnt/1
  Logical24/1 -> wr_cnt/1
  [wr_en] -> wr_cnt/2
  [rd_en] -> rd_cnt/2
  wr_cnt/1 -> AddSub/2
  Constant4/1 -> AddSub/1
  AddSub/1 -> Relational5/1
  Logical22/1 -> vect_cnt_rd/1
  vect_cnt_rd/1 -> Relational6/1, [vect_cnt_rd]
  [end_of_vector_rd] -> vect_cnt_rd/2
  Relational6/1 -> [last_acc_rd]
  [new_acc_wr] -> Logical22/2
  [rst] -> Logical22/1
  [new_acc_wr] -> Logical3/2
  [rst] -> Logical3/1
  Constant6/1 -> Logical1/8
  Constant7/1 -> Logical14/6
  [rst] -> tag_cnt/1
  [new_acc_wr] -> Logical23/2
  [rst] -> Logical23/1
  Logical23/1 -> vect_cnt_wr/1
  Logical16/1 -> Delay46/1
  [new_acc_wr] -> Logical24/2
  [rst] -> Logical24/1
  [new_acc_wr] -> Logical25/2
  [rst] -> Logical25/1
  [new_acc_wr] -> Register4/3
  Delay19/1 -> blank/1, [blank]
  [last_acc_wr] -> Delay45/1
  Delay45/1 -> Delay17/1
  Delay46/1 -> Delay18/1
  [mem_erase] -> Logical21/1
  Logical21/1 -> Delay19/1
  Delay44/1 -> Logical21/2
  [new_acc_wr] -> Delay43/1
  [erase_addr] -> Slice4/1
  Relational8/1 -> Logical19/2
  Constant9/1 -> Relational8/2
  Delay43/1 -> Logical19/3
  Logical19/1 -> error/1
  Slice4/1 -> Relational8/1
  Delay56/1 -> Logical19/1
  [first_acc_done] -> Delay56/1

== system s_b16a4x32kf/sys2/vacc/hmc_vacc/fifo_status ==
  out_fetch_valid : Inport
  out_fetch_empty : Inport  Port=2
  out_fetch_full : Inport  Port=3
  out_fetch_afull : Inport  Port=4
  out_rst : Inport  Port=5
  out_fifo_rd_en : Inport  Port=6
  out_rb_en : Inport  Port=7
  out_out_ack : Inport  Port=8
  out_output_full : Inport  Port=9
  out_output_over : Inport  Port=10
  out_input_empty : Inport  Port=11
  out_input_over : Inport  Port=12
  out_output_empty : Inport  Port=13
  assert_fetch_afull : xbsIndex_r4/Assert  assert_type=on  type_source=Explicitly  gui_display_data_type=Boolean  arith_type=Boolean  n_bits=1  bin_pt=0  preci_type=Single  exp_width=8  frac_width=24  assert_rate=off  rate_source=Explicitly  period=1  output_port=on  block_type=assert
  assert_fetch_empty : xbsIndex_r4/Assert  assert_type=on  type_source=Explicitly  gui_display_data_type=Boolean  arith_type=Boolean  n_bits=1  bin_pt=0  preci_type=Single  exp_width=8  frac_width=24  assert_rate=off  rate_source=Explicitly  period=1  output_port=on  block_type=assert
  assert_fetch_full : xbsIndex_r4/Assert  assert_type=on  type_source=Explicitly  gui_display_data_type=Boolean  arith_type=Boolean  n_bits=1  bin_pt=0  preci_type=Single  exp_width=8  frac_width=24  assert_rate=off  rate_source=Explicitly  period=1  output_port=on  block_type=assert
  assert_fetch_valid : xbsIndex_r4/Assert  assert_type=on  type_source=Explicitly  gui_display_data_type=Boolean  arith_type=Boolean  n_bits=1  bin_pt=0  preci_type=Single  exp_width=8  frac_width=24  assert_rate=off  rate_source=Explicitly  period=1  output_port=on  block_type=assert
  assert_fifo_rd_en : xbsIndex_r4/Assert  assert_type=on  type_source=Explicitly  gui_display_data_type=Boolean  arith_type=Boolean  n_bits=1  bin_pt=0  preci_type=Single  exp_width=8  frac_width=24  assert_rate=off  rate_source=Explicitly  period=1  output_port=on  block_type=assert
  assert_input_empty : xbsIndex_r4/Assert  assert_type=on  type_source=Explicitly  gui_display_data_type=Boolean  arith_type=Boolean  n_bits=1  bin_pt=0  preci_type=Single  exp_width=8  frac_width=24  assert_rate=off  rate_source=Explicitly  period=1  output_port=on  block_type=assert
  assert_input_over : xbsIndex_r4/Assert  assert_type=on  type_source=Explicitly  gui_display_data_type=Boolean  arith_type=Boolean  n_bits=1  bin_pt=0  preci_type=Single  exp_width=8  frac_width=24  assert_rate=off  rate_source=Explicitly  period=1  output_port=on  block_type=assert
  assert_out_ack : xbsIndex_r4/Assert  assert_type=on  type_source=Explicitly  gui_display_data_type=Boolean  arith_type=Boolean  n_bits=1  bin_pt=0  preci_type=Single  exp_width=8  frac_width=24  assert_rate=off  rate_source=Explicitly  period=1  output_port=on  block_type=assert
  assert_output_empty : xbsIndex_r4/Assert  assert_type=on  type_source=Explicitly  gui_display_data_type=Boolean  arith_type=Boolean  n_bits=1  bin_pt=0  preci_type=Single  exp_width=8  frac_width=24  assert_rate=off  rate_source=Explicitly  period=1  output_port=on  block_type=assert
  assert_output_full : xbsIndex_r4/Assert  assert_type=on  type_source=Explicitly  gui_display_data_type=Boolean  arith_type=Boolean  n_bits=1  bin_pt=0  preci_type=Single  exp_width=8  frac_width=24  assert_rate=off  rate_source=Explicitly  period=1  output_port=on  block_type=assert
  assert_output_over : xbsIndex_r4/Assert  assert_type=on  type_source=Explicitly  gui_display_data_type=Boolean  arith_type=Boolean  n_bits=1  bin_pt=0  preci_type=Single  exp_width=8  frac_width=24  assert_rate=off  rate_source=Explicitly  period=1  output_port=on  block_type=assert
  assert_rb_en : xbsIndex_r4/Assert  assert_type=on  type_source=Explicitly  gui_display_data_type=Boolean  arith_type=Boolean  n_bits=1  bin_pt=0  preci_type=Single  exp_width=8  frac_width=24  assert_rate=off  rate_source=Explicitly  period=1  output_port=on  block_type=assert
  assert_rst : xbsIndex_r4/Assert  assert_type=on  type_source=Explicitly  gui_display_data_type=Boolean  arith_type=Boolean  n_bits=1  bin_pt=0  preci_type=Single  exp_width=8  frac_width=24  assert_rate=off  rate_source=Explicitly  period=1  output_port=on  block_type=assert
  cast_gw : xbsIndex_r4/Convert  gui_display_data_type=Fixed-point  arith_type=Unsigned  n_bits=32  bin_pt=0  float_type=Single  exp_bits=8  fraction_bits=24  quantization=Truncate  overflow=Wrap  en=off  latency=1  pipeline=off  dbl_ovrd=off  block_type=convert
  concatenate : xbsIndex_r4/Concat  num_inputs=13  dbl_ovrd=off  block_type=concat
  io_delay : xbsIndex_r4/Delay  rst=off  infoeditControl=Selection of Reset will increase slice count due to use of real FFs and instead of SRLs  en=off  latency=0  reg_retiming=on  dbl_ovrd=off  block_type=delay
  reint{1..13} (13 alike) : xbsIndex_r4/Reinterpret  force_arith_type=on  arith_type=Unsigned  force_bin_pt=on  bin_pt=0  block_type=reinterpret
  s_b32a4x1kf_sys2_vacc_hmc_vacc_fifo_status_user_data_in : xbsIndex_r4/Gateway Out  inherit_from_input=off  hdl_port=on  rows=1  columns=1  UseAsDAC=off  DACChannel='1'  interface=None  automatic_assignment=on  address_offset=hex2dec('00')  intf_name=''  intf_description=''  timing_constraint=None  locs_specified=off  LOCs={}  io_standard={}  block_type=gatewayout
  sim_out : Terminator
  wires:
  concatenate/1 -> io_delay/1
  io_delay/1 -> cast_gw/1
  cast_gw/1 -> s_b32a4x1kf_sys2_vacc_hmc_vacc_fifo_status_user_data_in/1
  s_b32a4x1kf_sys2_vacc_hmc_vacc_fifo_status_user_data_in/1 -> sim_out/1
  out_fetch_valid/1 -> assert_fetch_valid/1
  assert_fetch_valid/1 -> reint1/1
  reint1/1 -> concatenate/1
  out_fetch_empty/1 -> assert_fetch_empty/1
  assert_fetch_empty/1 -> reint2/1
  reint2/1 -> concatenate/2
  out_fetch_full/1 -> assert_fetch_full/1
  assert_fetch_full/1 -> reint3/1
  reint3/1 -> concatenate/3
  out_fetch_afull/1 -> assert_fetch_afull/1
  assert_fetch_afull/1 -> reint4/1
  reint4/1 -> concatenate/4
  out_rst/1 -> assert_rst/1
  assert_rst/1 -> reint5/1
  reint5/1 -> concatenate/5
  out_fifo_rd_en/1 -> assert_fifo_rd_en/1
  assert_fifo_rd_en/1 -> reint6/1
  reint6/1 -> concatenate/6
  out_rb_en/1 -> assert_rb_en/1
  assert_rb_en/1 -> reint7/1
  reint7/1 -> concatenate/7
  out_out_ack/1 -> assert_out_ack/1
  assert_out_ack/1 -> reint8/1
  reint8/1 -> concatenate/8
  out_output_full/1 -> assert_output_full/1
  assert_output_full/1 -> reint9/1
  reint9/1 -> concatenate/9
  out_output_over/1 -> assert_output_over/1
  assert_output_over/1 -> reint10/1
  reint10/1 -> concatenate/10
  out_input_empty/1 -> assert_input_empty/1
  assert_input_empty/1 -> reint11/1
  reint11/1 -> concatenate/11
  out_input_over/1 -> assert_input_over/1
  assert_input_over/1 -> reint12/1
  reint12/1 -> concatenate/12
  out_output_empty/1 -> assert_output_empty/1
  assert_output_empty/1 -> reint13/1
  reint13/1 -> concatenate/13

== system s_b16a4x32kf/sys2/vacc/hmc_vacc/half_sel ==
  In1 : Inport
  Concat1 : xbsIndex_r4/Concat  num_inputs=3  dbl_ovrd=off  block_type=concat
      settings: block_version=10.1.3
  Constant3 : xbsIndex_r4/Constant  const=link  gui_display_data_type=Fixed-point  arith_type=Unsigned  n_bits=1  bin_pt=0  preci_type=Single  exp_width=8  frac_width=24  explicit_period=on  period=1  equ=P=C  opselect=C  inp2=PCIN>>17  opr=+  inp1=P  carry=CIN  dbl_ovrd=off  block_type=constant
  Slice1 : xbsIndex_r4/Slice  nbits=2  boolean_output=off  mode=Lower Bit Location + Width  bit1=96  base1=MSB of Input  bit0=0  base0=LSB of Input  dbl_ovrd=off  block_type=slice
      settings: block_version=9.2.01
  Slice5 : xbsIndex_r4/Slice  nbits=23  boolean_output=off  mode=Two Bit Locations  bit1=0  base1=MSB of Input  bit0=2  base0=LSB of Input  dbl_ovrd=off  block_type=slice
      settings: block_version=9.2.01
  Out1 : Outport
  wires:
  In1/1 -> Slice1/1, Slice5/1
  Slice5/1 -> Concat1/1
  Constant3/1 -> Concat1/2
  Slice1/1 -> Concat1/3
  Concat1/1 -> Out1/1

== system s_b16a4x32kf/sys2/vacc/hmc_vacc/half_sel1 ==
  In1 : Inport
  Concat1 : xbsIndex_r4/Concat  num_inputs=3  dbl_ovrd=off  block_type=concat
      settings: block_version=10.1.3
  Constant3 : xbsIndex_r4/Constant  const=link  gui_display_data_type=Fixed-point  arith_type=Unsigned  n_bits=1  bin_pt=0  preci_type=Single  exp_width=8  frac_width=24  explicit_period=on  period=1  equ=P=C  opselect=C  inp2=PCIN>>17  opr=+  inp1=P  carry=CIN  dbl_ovrd=off  block_type=constant
  Slice1 : xbsIndex_r4/Slice  nbits=2  boolean_output=off  mode=Lower Bit Location + Width  bit1=96  base1=MSB of Input  bit0=0  base0=LSB of Input  dbl_ovrd=off  block_type=slice
      settings: block_version=9.2.01
  Slice5 : xbsIndex_r4/Slice  nbits=23  boolean_output=off  mode=Two Bit Locations  bit1=0  base1=MSB of Input  bit0=2  base0=LSB of Input  dbl_ovrd=off  block_type=slice
      settings: block_version=9.2.01
  Out1 : Outport
  wires:
  In1/1 -> Slice1/1, Slice5/1
  Slice5/1 -> Concat1/1
  Constant3/1 -> Concat1/2
  Slice1/1 -> Concat1/3
  Concat1/1 -> Out1/1

== system s_b16a4x32kf/sys2/vacc/hmc_vacc/half_sel2 ==
  In1 : Inport
  Concat1 : xbsIndex_r4/Concat  num_inputs=3  dbl_ovrd=off  block_type=concat
      settings: block_version=10.1.3
  Constant3 : xbsIndex_r4/Constant  const=link  gui_display_data_type=Fixed-point  arith_type=Unsigned  n_bits=1  bin_pt=0  preci_type=Single  exp_width=8  frac_width=24  explicit_period=on  period=1  equ=P=C  opselect=C  inp2=PCIN>>17  opr=+  inp1=P  carry=CIN  dbl_ovrd=off  block_type=constant
  Slice1 : xbsIndex_r4/Slice  nbits=2  boolean_output=off  mode=Lower Bit Location + Width  bit1=96  base1=MSB of Input  bit0=0  base0=LSB of Input  dbl_ovrd=off  block_type=slice
      settings: block_version=9.2.01
  Slice5 : xbsIndex_r4/Slice  nbits=23  boolean_output=off  mode=Two Bit Locations  bit1=0  base1=MSB of Input  bit0=2  base0=LSB of Input  dbl_ovrd=off  block_type=slice
      settings: block_version=9.2.01
  Out1 : Outport
  wires:
  In1/1 -> Slice1/1, Slice5/1
  Slice5/1 -> Concat1/1
  Constant3/1 -> Concat1/2
  Slice1/1 -> Concat1/3
  Concat1/1 -> Out1/1
